simulink model "drive_thermal"  (R2026b)
settings: Solver=VariableStepAuto
undefined symbols (not defined in the file or in its folder): P
libraries: fl_lib x12, nesl_utility x5
settings Model: Creator=aomar  LastModifiedBy=aomar

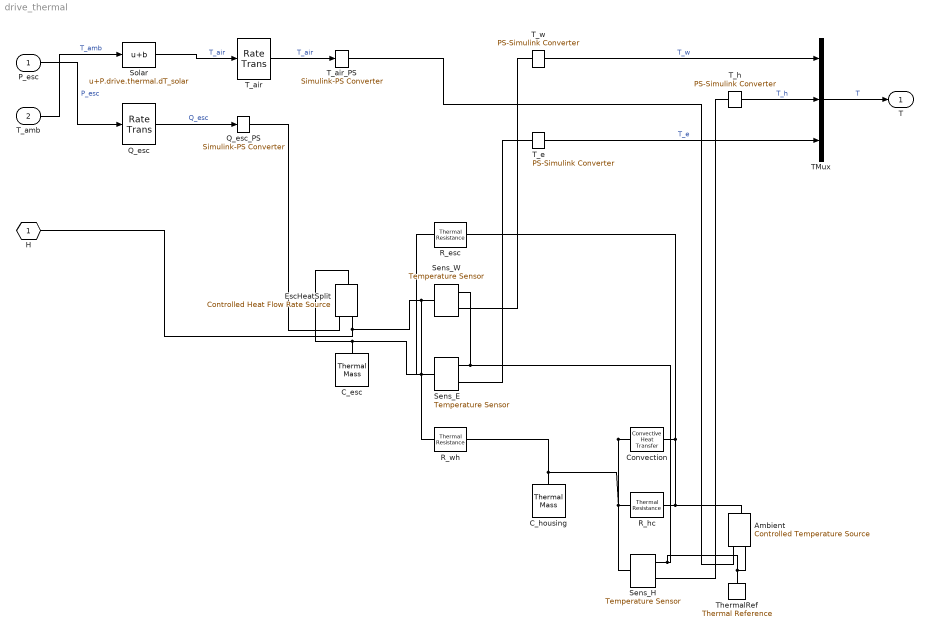
== system drive_thermal ==
  P_esc : Inport  OutDataTypeStr=double  SampleTime=P.drive.Ts_esc
  T_amb : Inport  Port=2  OutDataTypeStr=double  SampleTime=P.drive.Ts_esc
  Ambient : fl_lib/Thermal/Thermal Sources/Controlled Temperature Source
  C_esc : fl_lib/Thermal/Thermal Elements/Thermal Mass  mass_type=foundation.enum.constant_variable.constant  mass=P.drive.thermal.m_esc kg  sp_heat=P.drive.thermal.cp_esc J/(K*kg)  mass_min=1e-6 kg  num_ports=foundation.enum.numPorts2.one  m_specify=off  m_priority=High  m=1 kg  m_nominal_specify=off  m_nominal_value=1  m_nominal_unit=kg  T_specify=on  T_priority=High  T=P.drive.thermal.T_amb0 K  T_nominal_specify=off  T_nominal_value=1  T_nominal_unit=K  Q_specify=off  Q_priority=None  Q=0 W  Q_nominal_specify=off  Q_nominal_value=1  Q_nominal_unit=W
  C_housing : fl_lib/Thermal/Thermal Elements/Thermal Mass  mass_type=foundation.enum.constant_variable.constant  mass=P.drive.thermal.m_h kg  sp_heat=P.drive.thermal.cp_h J/(K*kg)  mass_min=1e-6 kg  num_ports=foundation.enum.numPorts2.one  m_specify=off  m_priority=High  m=1 kg  m_nominal_specify=off  m_nominal_value=1  m_nominal_unit=kg  T_specify=on  T_priority=High  T=P.drive.thermal.T_amb0 K  T_nominal_specify=off  T_nominal_value=1  T_nominal_unit=K  Q_specify=off  Q_priority=None  Q=0 W  Q_nominal_specify=off  Q_nominal_value=1  Q_nominal_unit=W
  Convection : fl_lib/Thermal/Thermal Elements/Convective Heat Transfer  thermal_type=foundation.enum.constant_variable.constant  area=P.drive.thermal.A_h m^2  heat_tr_coeff=P.drive.thermal.h_h W/(K*m^2)  min_heat_tr_coeff=1e-3 W/(K*m^2)  T_specify=off  T_priority=None  T=0 K  T_nominal_specify=off  T_nominal_value=1  T_nominal_unit=K  Q_specify=off  Q_priority=None  Q=0 W  Q_nominal_specify=off  Q_nominal_value=1  Q_nominal_unit=W
  EscHeatSplit : fl_lib/Thermal/Thermal Sources/Controlled Heat Flow Rate Source
  Q_esc : RateTransition  OutPortSampleTimeOpt=Inherit
  Q_esc_PS : nesl_utility/Simulink-PS Converter  PhysicalDomain=network_engine_domain  SubClassName=ps_input  LeftPortType=input  RightPortType=output  PseudoPeriodic=off  Frequencies=[]  NoiseDistribution=none  NoiseParameters=[]  Unit=W  AffineConversion=off  FilteringAndDerivatives=zero  SimscapeFilterOrder=1  InputFilterTimeConstant=0.001  UdotUserProvided=0
  R_esc : fl_lib/Thermal/Thermal Elements/Thermal Resistance  resistance=P.drive.thermal.R_esc K/W  T_specify=off  T_priority=None  T=0 K  T_nominal_specify=off  T_nominal_value=1  T_nominal_unit=K  Q_specify=off  Q_priority=None  Q=0 W  Q_nominal_specify=off  Q_nominal_value=1  Q_nominal_unit=W
  R_hc : fl_lib/Thermal/Thermal Elements/Thermal Resistance  resistance=P.drive.thermal.R_hc K/W  T_specify=off  T_priority=None  T=0 K  T_nominal_specify=off  T_nominal_value=1  T_nominal_unit=K  Q_specify=off  Q_priority=None  Q=0 W  Q_nominal_specify=off  Q_nominal_value=1  Q_nominal_unit=W
  R_wh : fl_lib/Thermal/Thermal Elements/Thermal Resistance  resistance=P.drive.thermal.R_wh K/W  T_specify=off  T_priority=None  T=0 K  T_nominal_specify=off  T_nominal_value=1  T_nominal_unit=K  Q_specify=off  Q_priority=None  Q=0 W  Q_nominal_specify=off  Q_nominal_value=1  Q_nominal_unit=W
  Sens_E : fl_lib/Thermal/Thermal Sensors/Temperature Sensor  temperature_measure=foundation.enum.MeasurementReference.difference
  Sens_H : fl_lib/Thermal/Thermal Sensors/Temperature Sensor  temperature_measure=foundation.enum.MeasurementReference.difference
  Sens_W : fl_lib/Thermal/Thermal Sensors/Temperature Sensor  temperature_measure=foundation.enum.MeasurementReference.difference
  Solar : Bias  Bias=P.drive.thermal.dT_solar  SaturateOnIntegerOverflow=off
  TMux : Mux  Inputs=3
  T_air : RateTransition  OutPortSampleTimeOpt=Inherit
  T_air_PS : nesl_utility/Simulink-PS Converter  PhysicalDomain=network_engine_domain  SubClassName=ps_input  LeftPortType=input  RightPortType=output  PseudoPeriodic=off  Frequencies=[]  NoiseDistribution=none  NoiseParameters=[]  Unit=K  AffineConversion=on  FilteringAndDerivatives=zero  SimscapeFilterOrder=1  InputFilterTimeConstant=0.001  UdotUserProvided=0
  T_e : nesl_utility/PS-Simulink Converter  PhysicalDomain=network_engine_domain  SubClassName=ps_output  LeftPortType=input  RightPortType=output  PseudoPeriodic=off  Frequencies=[]  VectorFormat=inherit  Unit=K  AffineConversion=on
  T_h : nesl_utility/PS-Simulink Converter  PhysicalDomain=network_engine_domain  SubClassName=ps_output  LeftPortType=input  RightPortType=output  PseudoPeriodic=off  Frequencies=[]  VectorFormat=inherit  Unit=K  AffineConversion=on
  T_w : nesl_utility/PS-Simulink Converter  PhysicalDomain=network_engine_domain  SubClassName=ps_output  LeftPortType=input  RightPortType=output  PseudoPeriodic=off  Frequencies=[]  VectorFormat=inherit  Unit=K  AffineConversion=on
  ThermalRef : fl_lib/Thermal/Thermal Elements/Thermal Reference
  H : PMIOPort  Side=Left  ConnectionType=Connection: foundation.thermal.thermal
  T : Outport  OutDataTypeStr=double
  wires:
  P_esc/1 -> Q_esc/1  "P_esc"
  T_amb/1 -> Solar/1  "T_amb"
  Solar/1 -> T_air/1  "T_air"
  Q_esc/1 -> Q_esc_PS/1  "Q_esc"
  T_air/1 -> T_air_PS/1  "T_air"
  T_w/1 -> TMux/1  "T_w"
  T_e/1 -> TMux/3  "T_e"
  T_h/1 -> TMux/2  "T_h"
  TMux/1 -> T/1  "T"
  connections:
  Convection/RConn1 -- R_esc/RConn1 -- R_hc/RConn1 -- Ambient/LConn1
  T_air_PS/RConn1 -- Ambient/RConn1
  Sens_E/RConn1 -- Sens_W/RConn1 -- Sens_H/RConn1 -- ThermalRef/LConn1 -- Ambient/RConn2
  C_housing/LConn1 -- R_wh/RConn1 -- R_hc/LConn1 -- Convection/LConn1 -- Sens_H/LConn1
  Q_esc_PS/RConn1 -- EscHeatSplit/RConn1
  T_e/LConn1 -- Sens_E/RConn2
  T_h/LConn1 -- Sens_H/RConn2
  T_w/LConn1 -- Sens_W/RConn2
  Sens_E/LConn1 -- R_esc/LConn1 -- C_esc/LConn1 -- EscHeatSplit/LConn1
  EscHeatSplit/RConn2 -- H/RConn1 -- Sens_W/LConn1 -- R_wh/LConn1
